simulink model "zad2"  (R2022b)
settings: Solver=FixedStepAuto  StartTime=0.0  StopTime=20.0  FixedStep=0.00001  RelTol=1e-3
model workspace (MAT data in the model file):
  K = 10
  T1 = 5
  T2 = 0.166666666667
settings Model: Creator=vandm  LastModifiedBy=vandm

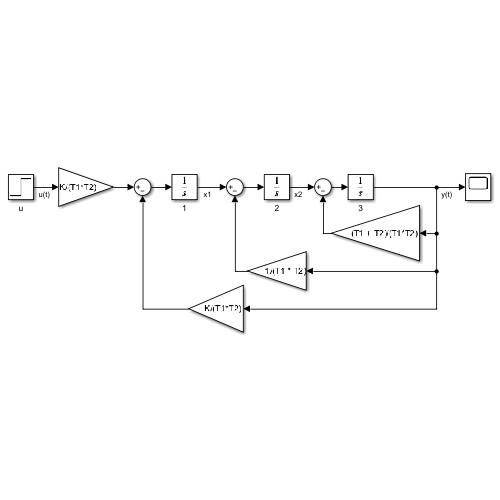
[thumbnail: Simulink's stored preview of the top-level diagram]
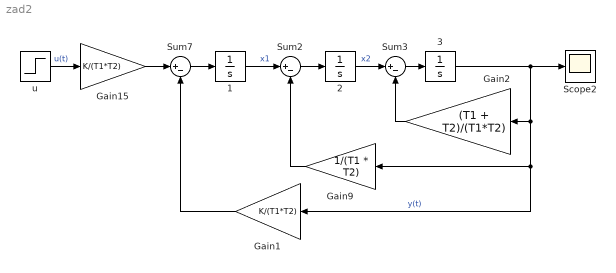
== system zad2 ==
  1 : Integrator  InitialCondition=1/(T1 * T2)
  2 : Integrator  InitialCondition=(T1 + T2)/(T1 * T2)
  3 : Integrator  InitialCondition=1
  Gain1 : Gain  Gain=K/(T1*T2)
  Gain15 : Gain  Gain=K/(T1*T2)
  Gain2 : Gain  Gain=(T1 + T2)/(T1*T2)
  Gain9 : Gain  Gain=1/(T1 * T2)
  Scope2 : Scope
  Sum2 : Sum  Inputs=|+-
  Sum3 : Sum  Inputs=|+-
  Sum7 : Sum  Inputs=|+-
  u : Step  Time=0  After=0  SampleTime=0
  wires:
  Gain1/1 -> Sum7/2
  1/1 -> Sum2/1  "x1"
  Gain9/1 -> Sum2/2
  u/1 -> Gain15/1  "u(t)"
  Sum7/1 -> 1/1
  Sum2/1 -> 2/1
  2/1 -> Sum3/1  "x2"
  Gain2/1 -> Sum3/2
  3/1 -> Gain2/1, Gain9/1, Gain1/1, Scope2/1  "y(t)"
  Sum3/1 -> 3/1
  Gain15/1 -> Sum7/1
